simulink library "casper_library_flow_control"  (Simulink 7.2)
settings: Solver=ode45  SolverMode=SingleTasking  StartTime=0.0  StopTime=10.0  RelTol=1e-3
libraries: xbsIndex_r4 x22, casper_library_flow_control x16
settings Model: Creator=mdexter  LastModifiedBy=mdexter

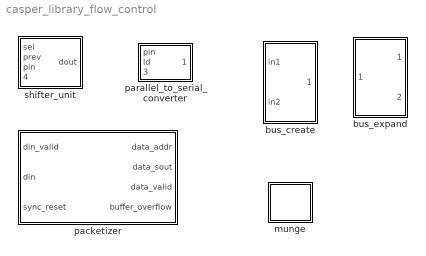
== system casper_library_flow_control ==
  bus_create : Subsystem  mask(bus_create){inputNum=2}
      mask prompts: inputNum "Number of inputs:"
      mask init:
      | bus_create_init(gcb,...
      |     'inputNum', inputNum);
  bus_expand : Subsystem  mask(bus_expand){mode=divisions of equal size, outputNum=2, outputWidth=16, outputBinaryPt=0, outputArithmeticType=0, show_format=off, outputToWorkspace=off, variablePrefix=out, outputToModelAsWell=on}
      mask prompts: outputNum "Number of outputs:"; outputWidth "Output width:"; outputBinaryPt "Output binary point position:"; outputArithmeticType "Output arithmetic type (ufix=0, fix=1, bool=2):"; show_format "Print format string?"; outputToWorkspace "Output to workspace?"; variablePrefix "Variable name prefix:"; outputToModelAsWell "Output to model as well?"
      mask help:
      | Expands a 'bus' made using a bus_create or Xilinx
      | concat block.
      | The input will be divided into the specified number
      | of outputs with the specified arithmetic types.
      | Divisions are made from most significant bit.
      mask init:
      | bus_expand_init(gcb,...
      |     'mode', mode, ...
      |     'outputNum', outputNum, ...
      |     'outputWidth', outputWidth, ...
      |     'outputBinaryPt', outputBinaryPt, ...
      |     'outputArithmeticType', outputArithmeticType, ...
      |     'show_format', show_format, ...
      |     'outputToWorkspace', outputToWorkspace, ...
      |     'variablePrefix', variablePrefix, ...
      |     'outputToModelAsWell', outputToModelAsWell);
      settings: AttributesFormatString=2 outputs
      mask StyleString: popup(divisions of equal size|divisions of arbitrary size),edit,edit,edit,edit,checkbox,checkbox,edit,checkbox
      mask CallbackString: bus_expand_callback();||bus_expand_callback();||||bus_expand_callback();||
  munge : Subsystem  mask(munge){divisions=0, div_size=1, order=0, arith_type_out=Unsigned, bin_pt_out=0}
      mask prompts: divisions "Number of divisions"; div_size "Division size (bits)"; order "Division packing order"; arith_type_out "Output arithmetic type"; bin_pt_out "Output binary point"
      mask help: Splits an input bus into the specified number of divisions and then recombines them in the order specified (most significant division = 0,least = number divisions-1)
      mask init:
      | munge_init(gcb, ...
      |     'divisions', divisions, ...
      |     'div_size', div_size, ...
      |     'order', order, ...
      |     'arith_type_out', arith_type_out, ...
      |     'bin_pt_out', bin_pt_out);
      mask StyleString: edit,edit,edit,popup(Unsigned|Signed  (2's comp)|Floating-point),edit
  packetizer : Subsystem  mask(packetizer){pin_width=512, sout_width=64, fifo_depth=64, total_words=64}
      mask prompts: pin_width "Parallel Input Width"; sout_width "Serial Output Width"; fifo_depth "FIFO depth"; total_words "Total number of data points"
      mask help:
      | This block is intended to serialize data that is 'bursty', that is,
      | the average data rate is small but per cycle the data is highly
      | parallel and can contain many points simultaneously.  This situation
      | is common with the streaming CASPER FFTs and related blocks.
      |
      | The serialization buffers the data when valid and independently
      | serializes the data when the buffer is non-empty.  For convenience, the
      | data is counted as it is serialized and signals exist to indicate
      | that the serial output is valid or that a buffer overflow has occured.  The
      | block will not stop in the case of an overflow, and the overflow
      | signal is not held high after it occurs.
      |
      | For example usage, see 'roach_spec_2adc_borph' in 'SVNROOT/trunk/projects/roach_spec/'
      | or the test case in 'SVNROOT/trunk/mlib_devel_10_1/Tests/packetizer_test.mdl'
      |
      | For extended documentation, please see the CASPER wiki
      mask init:
      | packetizer_init(gcb, 'pin_width', pin_width, 'sout_width', sout_width, 'total_words', total_words, 'fifo_depth', fifo_depth)
      | % packetizer_init(gcb, ...
      | %     'pin_width', pin_width, ...
      | %     'sout_width', sout_width, ...
      | %   %  'fifo_depth', fifo_depth, ...
      | %     'total_words', total_words);
      settings: AttributesFormatString=|
      | Parallel Input Width: 512
      | Serial Output Width: 64
      mask StyleString: edit,edit,popup(16|32|64|128|256|512|1K|2K|4K|8K|16K|32K|64K),edit
  parallel_to_serial_converter : Subsystem  mask(parallel_to_serial_converter){pin_width=128, sout_width=16}
      mask prompts: pin_width "Parallel Input Width"; sout_width "Serial Output Width"
      mask help:
      | This block takes as input a parallel bus of specified width.
      | When the load signal 'ld' is asserted, this data is broken into
      | pieces of width specified by the serial output width and
      | stored into different registers chained to form a shift register.
      | If the 'shift' input is subsequently asserted, the shift register
      | returns as output a new piece of data of width sout_width.  This data
      | is the next least significant piece of the original bus.  The converter
      | serializes SMALL ENDIAN.
      |
      | Note that the load operation automatically loads the least significant
      | bits into the register closest to the output, so the first 'shift'
      | assertion changes the data output from bits [sout_width-1:0] to
      | bits [2*sout_width-1:sout_width].
      mask init:
      | parallel_to_serial_converter_init(gcb, ...
      |     'pin_width', pin_width, ...
      |     'sout_width', sout_width);
  shifter_unit : Subsystem  mask(shifter_unit){data_width=16, pin_offset=0}
      mask prompts: data_width "Data Width"; pin_offset "pin offset"
      mask help:
      | This block is simply a wrapper for a register with a multiplexer on the input.
      | Please see the documenation for the 'parallel_to_serial_converter'.

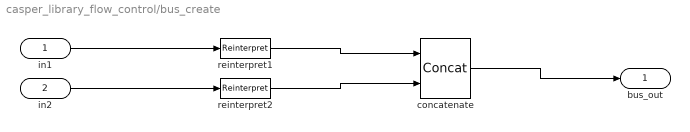
== system casper_library_flow_control/bus_create ==
  in1 : Inport
  in2 : Inport  Port=2
  concatenate : xbsIndex_r4/Concat  num_inputs=2  dbl_ovrd=off  block_type=concat
  reinterpret1 : xbsIndex_r4/Reinterpret  force_arith_type=on  arith_type=Unsigned  force_bin_pt=on  bin_pt=0  block_type=reinterpret
      settings: infoedit="Changes signal type without altering the binary representation.   You can changed the signal between signed and unsigned, and relocate the binary point.<br><br>Hardware notes: In hardware this block costs nothing.<br><br>Example:  Suppose the input is 6 bits wide, signed, with 2 fractional bits, and the output is forced to unsigned with 0 fractional bits.  Then an input of -2.0 (1110.00 in binary 2's complement) becomes an output of 56 (111000 in binary)."
  reinterpret2 : xbsIndex_r4/Reinterpret  force_arith_type=on  arith_type=Unsigned  force_bin_pt=on  bin_pt=0  block_type=reinterpret
      settings: infoedit="Changes signal type without altering the binary representation.   You can changed the signal between signed and unsigned, and relocate the binary point.<br><br>Hardware notes: In hardware this block costs nothing.<br><br>Example:  Suppose the input is 6 bits wide, signed, with 2 fractional bits, and the output is forced to unsigned with 0 fractional bits.  Then an input of -2.0 (1110.00 in binary 2's complement) becomes an output of 56 (111000 in binary)."
  bus_out : Outport
  wires:
  reinterpret2/1 -> concatenate/2
  in2/1 -> reinterpret2/1
  reinterpret1/1 -> concatenate/1
  in1/1 -> reinterpret1/1
  concatenate/1 -> bus_out/1

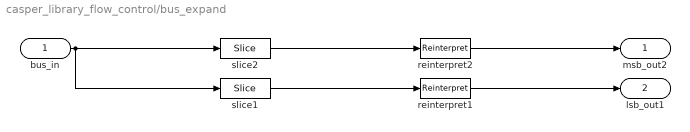
== system casper_library_flow_control/bus_expand ==
  bus_in : Inport
  reinterpret1 : xbsIndex_r4/Reinterpret  force_arith_type=on  arith_type=Unsigned  force_bin_pt=on  bin_pt=0  block_type=reinterpret
  reinterpret2 : xbsIndex_r4/Reinterpret  force_arith_type=on  arith_type=Unsigned  force_bin_pt=on  bin_pt=0  block_type=reinterpret
  slice1 : xbsIndex_r4/Slice  nbits=16  boolean_output=off  mode=Upper Bit Location + Width  bit1=-16  base1=MSB of Input  bit0=0  base0=LSB of Input  dbl_ovrd=off  block_type=slice
  slice2 : xbsIndex_r4/Slice  nbits=16  boolean_output=off  mode=Upper Bit Location + Width  bit1=0  base1=MSB of Input  bit0=0  base0=LSB of Input  dbl_ovrd=off  block_type=slice
  msb_out2 : Outport
  lsb_out1 : Outport  Port=2
  wires:
  bus_in/1 -> slice2/1, slice1/1
  slice2/1 -> reinterpret2/1
  reinterpret2/1 -> msb_out2/1
  slice1/1 -> reinterpret1/1
  reinterpret1/1 -> lsb_out1/1

== system casper_library_flow_control/munge ==

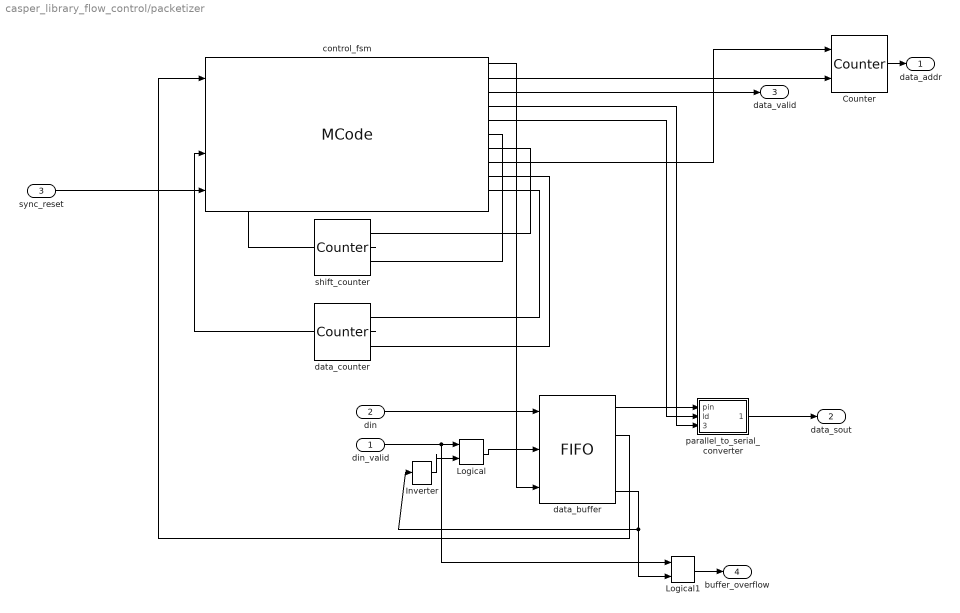
== system casper_library_flow_control/packetizer ==
  din_valid : Inport
  din : Inport  Port=2
  sync_reset : Inport  Port=3
  Counter : xbsIndex_r4/Counter  cnt_type=Free Running  cnt_to=Inf  operation=Up  start_count=0  cnt_by_val=1  arith_type=Unsigned  n_bits=11  bin_pt=0  load_pin=off  rst=on  en=on  explicit_period=on  period=1  dbl_ovrd=off  use_behavioral_HDL=off  implementation=Fabric  use_rpm=off  block_type=counter
  Inverter : xbsIndex_r4/Inverter  en=off  latency=0  dbl_ovrd=off  block_type=inv
  Logical : xbsIndex_r4/Logical  logical_function=AND  inputs=2  en=off  latency=0  precision=Full  arith_type=Unsigned  n_bits=16  bin_pt=0  align_bp=on  dbl_ovrd=off  block_type=logical
  Logical1 : xbsIndex_r4/Logical  logical_function=AND  inputs=2  en=off  latency=0  precision=Full  arith_type=Unsigned  n_bits=16  bin_pt=0  align_bp=on  dbl_ovrd=off  block_type=logical
  control_fsm : xbsIndex_r4/MCode  mfname=packetizer_fsm  explicit_period=on  period=1  inputsTable={'boundInpExpr'=>['','','7','',' 63 ',''],'inputs'=>['fifo_empty','shift_count','data_per_word','data_count','n_words','sync_reset']}  outputsTable={'outputs'=>['fifo_re','bram_addr_en','bram_we','serializer_shift','serializer_ld','shift_count_en','shift_count_rst','bram_addr_rst','data_count_en','data_count_rst'],'suppressOut'=>['off','off','off','off','off','off','off','off','off','off']}  dbl_ovrd=off  enable_stdout=off  enable_debug=off  suppress_output=1  defparams={'data_per_word',7, 'n_words', 63 }  hide_port_list={}  block_type=mcode
      settings: block_version=10.1.3
  data_buffer : xbsIndex_r4/FIFO  mem_type=Block RAM  performance_options=Standard_FIFO  infoedit1=Available only for V4, V5, V6, V7, K7, A7 and Zynq devices.  embedded_registers=off  depth=64  percent_nbits=1  rst=off  en=off  use_dcount=off  use_percent_full_port=on  use_almost_empty=off  almost_empty_thresh=2  use_almost_full=off  almost_full_thresh=14  dbl_ovrd=off  explicit_period=off  block_type=fifo
      settings: block_version=10.1.3
  data_counter : xbsIndex_r4/Counter  cnt_type=Free Running  cnt_to=Inf  operation=Up  start_count=0  cnt_by_val=1  arith_type=Unsigned  n_bits=7  bin_pt=0  load_pin=off  rst=on  en=on  explicit_period=on  period=1  dbl_ovrd=off  use_behavioral_HDL=off  implementation=Fabric  use_rpm=off  block_type=counter
  parallel_to_serial_converter : Subsystem  AncestorBlock=casper_library_flow_control/parallel_to_serial_converter  mask(parallel_to_serial_converter){pin_width=512, sout_width=64}
      mask prompts: pin_width "Parallel Input Width"; sout_width "Serial Output Width"
      mask help:
      | This block takes as input a parallel bus of specified width.
      | When the load signal 'ld' is asserted, this data is broken into
      | pieces of width specified by the serial output width and
      | stored into different registers chained to form a shift register.
      | If the 'shift' input is subsequently asserted, the shift register
      | returns as output a new piece of data of width sout_width.  This data
      | is the next least significant piece of the original bus.  The converter
      | serializes SMALL ENDIAN.
      |
      | Note that the load operation automatically loads the least significant
      | bits into the register closest to the output, so the first 'shift'
      | assertion changes the data output from bits [sout_width-1:0] to
      | bits [2*sout_width-1:sout_width].
      mask init:
      | parallel_to_serial_converter_init(gcb, ...
      |     'pin_width', pin_width, ...
      |     'sout_width', sout_width);
  shift_counter : xbsIndex_r4/Counter  cnt_type=Free Running  cnt_to=Inf  operation=Up  start_count=0  cnt_by_val=1  arith_type=Unsigned  n_bits=4  bin_pt=0  load_pin=off  rst=on  en=on  explicit_period=on  period=1  dbl_ovrd=off  use_behavioral_HDL=off  implementation=Fabric  use_rpm=off  block_type=counter
  data_addr : Outport
  data_sout : Outport  Port=2
  data_valid : Outport  Port=3
  buffer_overflow : Outport  Port=4
  wires:
  Logical1/1 -> buffer_overflow/1
  data_buffer/4 -> Logical1/2, Inverter/1
  Inverter/1 -> Logical/2
  din_valid/1 -> Logical1/1, Logical/1
  Logical/1 -> data_buffer/2
  data_buffer/1 -> parallel_to_serial_converter/1(pin)
  control_fsm/1 -> data_buffer/3
  control_fsm/4 -> parallel_to_serial_converter/3(shift)
  control_fsm/5 -> parallel_to_serial_converter/2(ld)
  control_fsm/3 -> data_valid/1
  din/1 -> data_buffer/1
  parallel_to_serial_converter/1(sout) -> data_sout/1
  control_fsm/6 -> shift_counter/2
  shift_counter/1 -> control_fsm/2
  control_fsm/7 -> shift_counter/1
  data_buffer/2 -> control_fsm/1
  Counter/1 -> data_addr/1
  control_fsm/2 -> Counter/2
  control_fsm/8 -> Counter/1
  control_fsm/9 -> data_counter/2
  data_counter/1 -> control_fsm/3
  sync_reset/1 -> control_fsm/4
  control_fsm/10 -> data_counter/1

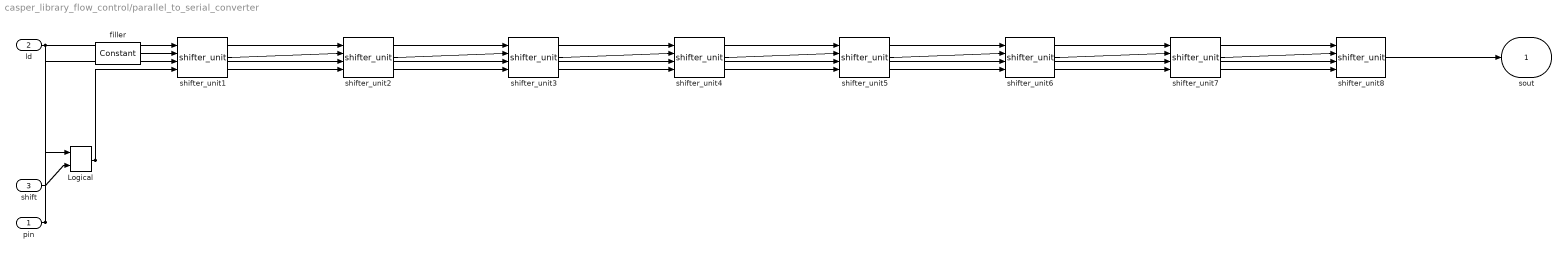
== system casper_library_flow_control/parallel_to_serial_converter ==
  pin : Inport
  ld : Inport  Port=2
  shift : Inport  Port=3
  Logical : xbsIndex_r4/Logical  logical_function=OR  inputs=2  en=off  latency=0  precision=Full  arith_type=Unsigned  n_bits=16  bin_pt=0  align_bp=on  dbl_ovrd=off  block_type=logical
  filler : xbsIndex_r4/Constant  const=0  gui_display_data_type=Fixed-point  arith_type=Unsigned  n_bits=sout_width  bin_pt=0  preci_type=Single  exp_width=8  frac_width=24  explicit_period=on  period=1  equ=P=C  opselect=C  inp2=PCIN>>17  opr=+  inp1=P  carry=CIN  dbl_ovrd=off  block_type=constant
  shifter_unit1 : casper_library_flow_control/shifter_unit  data_width=16  pin_offset=0
  shifter_unit2 : casper_library_flow_control/shifter_unit  data_width=16  pin_offset=16
  shifter_unit3 : casper_library_flow_control/shifter_unit  data_width=16  pin_offset=32
  shifter_unit4 : casper_library_flow_control/shifter_unit  data_width=16  pin_offset=48
  shifter_unit5 : casper_library_flow_control/shifter_unit  data_width=16  pin_offset=64
  shifter_unit6 : casper_library_flow_control/shifter_unit  data_width=16  pin_offset=80
  shifter_unit7 : casper_library_flow_control/shifter_unit  data_width=16  pin_offset=96
  shifter_unit8 : casper_library_flow_control/shifter_unit  data_width=16  pin_offset=112
  sout : Outport
  wires:
  shifter_unit8/1 -> sout/1
  shifter_unit7/1 -> shifter_unit8/2
  shifter_unit6/1 -> shifter_unit7/2
  shifter_unit5/1 -> shifter_unit6/2
  shifter_unit4/1 -> shifter_unit5/2
  shifter_unit3/1 -> shifter_unit4/2
  shifter_unit2/1 -> shifter_unit3/2
  shifter_unit1/1 -> shifter_unit2/2
  Logical/1 -> shifter_unit8/4, shifter_unit7/4, shifter_unit6/4, shifter_unit5/4, shifter_unit4/4, shifter_unit3/4, shifter_unit2/4, shifter_unit1/4
  pin/1 -> shifter_unit8/3, shifter_unit7/3, shifter_unit6/3, shifter_unit5/3, shifter_unit4/3, shifter_unit3/3, shifter_unit2/3, shifter_unit1/3
  filler/1 -> shifter_unit1/2
  shift/1 -> Logical/2
  ld/1 -> shifter_unit8/1, shifter_unit7/1, shifter_unit6/1, shifter_unit5/1, shifter_unit4/1, shifter_unit3/1, shifter_unit2/1, shifter_unit1/1, Logical/1

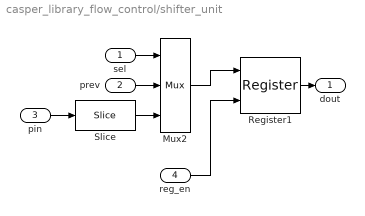
== system casper_library_flow_control/shifter_unit ==
  sel : Inport
  prev : Inport  Port=2
  pin : Inport  Port=3
  reg_en : Inport  Port=4
  Mux2 : xbsIndex_r4/Mux  inputs=2  en=off  latency=0  precision=Full  arith_type=Unsigned  n_bits=16  bin_pt=14  quantization=Truncate  overflow=Wrap  dbl_ovrd=off  block_type=mux
  Register1 : xbsIndex_r4/Register  init=0  rst=off  en=on  dbl_ovrd=off  block_type=register
  Slice : xbsIndex_r4/Slice  nbits=data_width  boolean_output=off  mode=Lower Bit Location + Width  bit1=0  base1=MSB of Input  bit0=pin_offset  base0=LSB of Input  dbl_ovrd=off  block_type=slice
      settings: infoedit="Extracts a given range of bits from each input sample and presents it at the output.  The output type is ordinarily unsigned with binary point at zero, but can be Boolean when the slice is one bit wide.<P><P>Hardware notes: In hardware this block costs nothing."  block_version=10.1.3
  dout : Outport
  wires:
  reg_en/1 -> Register1/2
  Mux2/1 -> Register1/1
  Register1/1 -> dout/1
  Slice/1 -> Mux2/3
  sel/1 -> Mux2/1
  prev/1 -> Mux2/2
  pin/1 -> Slice/1

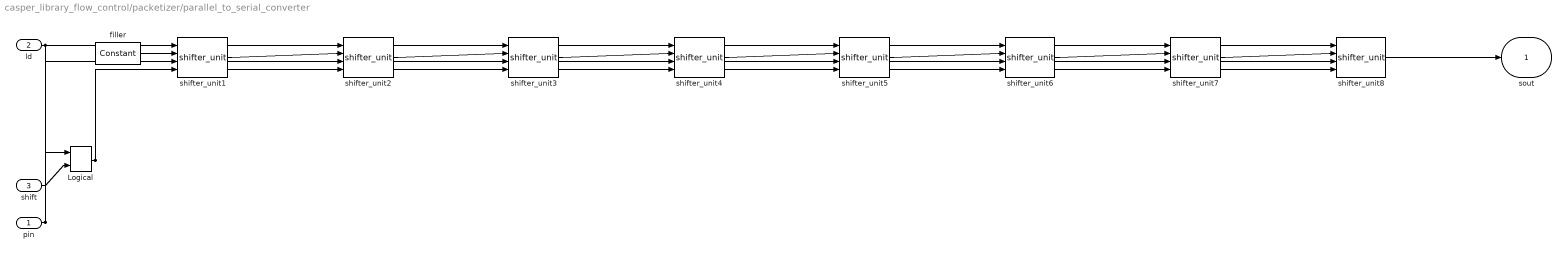
== system casper_library_flow_control/packetizer/parallel_to_serial_converter ==
  pin : Inport
  ld : Inport  Port=2
  shift : Inport  Port=3
  Logical : xbsIndex_r4/Logical  logical_function=OR  inputs=2  en=off  latency=0  precision=Full  arith_type=Unsigned  n_bits=16  bin_pt=0  align_bp=on  dbl_ovrd=off  block_type=logical
  filler : xbsIndex_r4/Constant  const=0  gui_display_data_type=Fixed-point  arith_type=Unsigned  n_bits=sout_width  bin_pt=0  preci_type=Single  exp_width=8  frac_width=24  explicit_period=on  period=1  equ=P=C  opselect=C  inp2=PCIN>>17  opr=+  inp1=P  carry=CIN  dbl_ovrd=off  block_type=constant
  shifter_unit1 : casper_library_flow_control/shifter_unit  data_width=64  pin_offset=0
  shifter_unit2 : casper_library_flow_control/shifter_unit  data_width=64  pin_offset=64
  shifter_unit3 : casper_library_flow_control/shifter_unit  data_width=64  pin_offset=128
  shifter_unit4 : casper_library_flow_control/shifter_unit  data_width=64  pin_offset=192
  shifter_unit5 : casper_library_flow_control/shifter_unit  data_width=64  pin_offset=256
  shifter_unit6 : casper_library_flow_control/shifter_unit  data_width=64  pin_offset=320
  shifter_unit7 : casper_library_flow_control/shifter_unit  data_width=64  pin_offset=384
  shifter_unit8 : casper_library_flow_control/shifter_unit  data_width=64  pin_offset=448
  sout : Outport
  wires:
  shifter_unit8/1 -> sout/1
  shifter_unit7/1 -> shifter_unit8/2
  shifter_unit6/1 -> shifter_unit7/2
  shifter_unit5/1 -> shifter_unit6/2
  shifter_unit4/1 -> shifter_unit5/2
  shifter_unit3/1 -> shifter_unit4/2
  shifter_unit2/1 -> shifter_unit3/2
  shifter_unit1/1 -> shifter_unit2/2
  Logical/1 -> shifter_unit8/4, shifter_unit7/4, shifter_unit6/4, shifter_unit5/4, shifter_unit4/4, shifter_unit3/4, shifter_unit2/4, shifter_unit1/4
  pin/1 -> shifter_unit8/3, shifter_unit7/3, shifter_unit6/3, shifter_unit5/3, shifter_unit4/3, shifter_unit3/3, shifter_unit2/3, shifter_unit1/3
  filler/1 -> shifter_unit1/2
  shift/1 -> Logical/2
  ld/1 -> shifter_unit8/1, shifter_unit7/1, shifter_unit6/1, shifter_unit5/1, shifter_unit4/1, shifter_unit3/1, shifter_unit2/1, shifter_unit1/1, Logical/1
